simulink model "afe_rst_ctrl"  (R2026b)
settings: Solver=ode23t  StopTime=param.sim.simlength  FixedStep=tc  MaxStep=param.glb_time.tc  RelTol=1e-4
values from neighbouring files (symbols this model uses):
  param = add_template_extras(param, options)    [init_model.m]
undefined symbols (not defined in the file or in its folder): magnitude
libraries: fl_lib x181, nesl_utility x97, igbt_simple_2th_lib x6, afe_uvw_ctrl x5, discrete_time_low_pass_filter x2, threephase_inductor_lib x1, dclink_for_two_levels x1, three_phase_pwm_modulator x1, three_phase_inverter_ideal_switch_based_model x1, three_phase_inverter_mosfet_based_with_thermal_model x1, ee_lib x1, three_phase_voltage_with_frt_emulator_mfcn x1
(part 2 of 6)

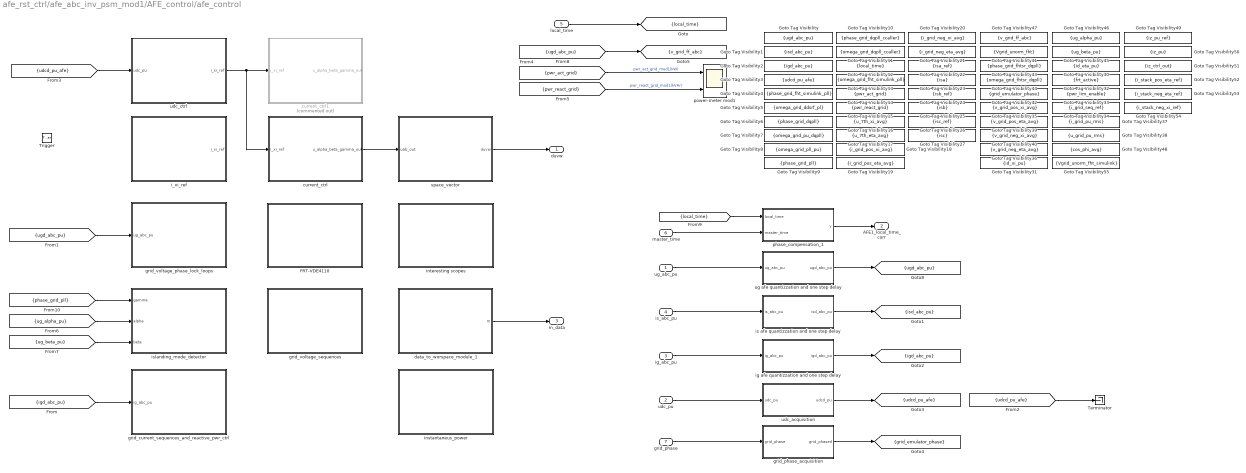
== system afe_rst_ctrl/afe_abc_inv_psm_mod1/AFE_control/afe_control ==
  ug_abc_pu : Inport
  udc_pu : Inport  Port=2
  ig_abc_pu : Inport  Port=3
  is_abc_pu : Inport  Port=4
  local_time : Inport  Port=5
  master_time : Inport  Port=6
  grid_phase : Inport  Port=7
  Trigger : TriggerPort  VariantControl=(inherit)  PortDimensions=1
  FRT-VDE4110 : Subsystem
  Goto Tag Visibility : GotoTagVisibility  GotoTag=ugd_abc_pu
  Goto Tag Visibility1 : GotoTagVisibility  GotoTag=isd_abc_pu
  Goto Tag Visibility10 : GotoTagVisibility  GotoTag=phase_grid_dqpll_ccaller
  Goto Tag Visibility11 : GotoTagVisibility  GotoTag=omega_grid_dqpll_ccaller
  Goto Tag Visibility12 : GotoTagVisibility  GotoTag=local_time
  Goto Tag Visibility13 : GotoTagVisibility  GotoTag=omega_grid_fht_simulink_pll
  Goto Tag Visibility14 : GotoTagVisibility  GotoTag=pwr_act_grid
  Goto Tag Visibility15 : GotoTagVisibility  GotoTag=pwr_react_grid
  Goto Tag Visibility16 : GotoTagVisibility  GotoTag=u_7th_xi_avg
  Goto Tag Visibility17 : GotoTagVisibility  GotoTag=u_7th_eta_avg
  Goto Tag Visibility18 : GotoTagVisibility  GotoTag=i_grid_pos_xi_avg
  Goto Tag Visibility19 : GotoTagVisibility  GotoTag=i_grid_pos_eta_avg
  Goto Tag Visibility2 : GotoTagVisibility  GotoTag=igd_abc_pu
  Goto Tag Visibility20 : GotoTagVisibility  GotoTag=i_grid_neg_xi_avg
  Goto Tag Visibility21 : GotoTagVisibility  GotoTag=i_grid_neg_eta_avg
  Goto Tag Visibility22 : GotoTagVisibility  GotoTag=isa_ref
  Goto Tag Visibility23 : GotoTagVisibility  GotoTag=isa
  Goto Tag Visibility24 : GotoTagVisibility  GotoTag=isb_ref
  Goto Tag Visibility25 : GotoTagVisibility  GotoTag=isb
  Goto Tag Visibility26 : GotoTagVisibility  GotoTag=isc_ref
  Goto Tag Visibility27 : GotoTagVisibility  GotoTag=isc
  Goto Tag Visibility3 : GotoTagVisibility  GotoTag=udcd_pu_afe
  Goto Tag Visibility30 : GotoTagVisibility  GotoTag=id_eta_pu
  Goto Tag Visibility31 : GotoTagVisibility  GotoTag=id_xi_pu
  Goto Tag Visibility32 : GotoTagVisibility  GotoTag=frt_active
  Goto Tag Visibility33 : GotoTagVisibility  GotoTag=pwr_lim_enable
  Goto Tag Visibility34 : GotoTagVisibility  GotoTag=i_grid_seq_ref
  Goto Tag Visibility35 : GotoTagVisibility  GotoTag=v_grid_pos_xi_avg
  Goto Tag Visibility36 : GotoTagVisibility  GotoTag=v_grid_neg_eta_avg
  Goto Tag Visibility37 : GotoTagVisibility  GotoTag=i_grid_pu_rms
  Goto Tag Visibility38 : GotoTagVisibility  GotoTag=u_grid_pu_rms
  Goto Tag Visibility39 : GotoTagVisibility  GotoTag=v_grid_pos_eta_avg
  Goto Tag Visibility4 : GotoTagVisibility  GotoTag=phase_grid_fht_simulink_pll
  Goto Tag Visibility40 : GotoTagVisibility  GotoTag=v_grid_neg_xi_avg
  Goto Tag Visibility41 : GotoTagVisibility  GotoTag=Vgrid_unorm_fht
  Goto Tag Visibility42 : GotoTagVisibility  GotoTag=grid_emulator_phase
  Goto Tag Visibility43 : GotoTagVisibility  GotoTag=phase_grid_fhtsr_dqpll
  Goto Tag Visibility44 : GotoTagVisibility  GotoTag=omega_grid_fhtsr_dqpll
  Goto Tag Visibility45 : GotoTagVisibility  GotoTag=ug_beta_pu
  Goto Tag Visibility46 : GotoTagVisibility  GotoTag=ug_alpha_pu
  Goto Tag Visibility47 : GotoTagVisibility  GotoTag=v_grid_ff_abc
  Goto Tag Visibility48 : GotoTagVisibility  GotoTag=cos_phi_avg
  Goto Tag Visibility49 : GotoTagVisibility  GotoTag=iz_pu_ref
  Goto Tag Visibility5 : GotoTagVisibility  GotoTag=omega_grid_ddsrf_pl
  Goto Tag Visibility50 : GotoTagVisibility  GotoTag=iz_pu
  Goto Tag Visibility51 : GotoTagVisibility  GotoTag=iz_ctrl_out
  Goto Tag Visibility52 : GotoTagVisibility  GotoTag=i_stack_pos_eta_ref
  Goto Tag Visibility53 : GotoTagVisibility  GotoTag=i_stack_neg_eta_ref
  Goto Tag Visibility54 : GotoTagVisibility  GotoTag=i_stack_neg_xi_ref
  Goto Tag Visibility55 : GotoTagVisibility  GotoTag=Vgrid_unorm_fht_simulink
  Goto Tag Visibility6 : GotoTagVisibility  GotoTag=phase_grid_dqpll
  Goto Tag Visibility7 : GotoTagVisibility  GotoTag=omega_grid_pu_dqpll
  Goto Tag Visibility8 : GotoTagVisibility  GotoTag=omega_grid_pll_pu
  Goto Tag Visibility9 : GotoTagVisibility  GotoTag=phase_grid_pll
  Terminator : Terminator
  current_ctrl : Subsystem
  current_ctrl1 : Subsystem  Commented=on
  data_to_worspace_module_1 : Subsystem
  grid_current_sequences_and_reactive_pwr_ctrl : Subsystem
  grid_phase_acquisition : Subsystem
  grid_voltage_phase_lock_loops : Subsystem
  grid_voltage_sequences : Subsystem
  i_xi_ref : Subsystem
  ig afe quantizzation and one step delay : Subsystem
  instantaneus_power : Subsystem
  interesting scopes : Subsystem
  is afe quantizzation and one step delay : Subsystem
  islanding_mode_detector : Subsystem
  phase_compensation_1 : Subsystem
  power-meter mod1 : Scope  NumInputPorts=2
      settings: ActiveDisplayYMinimum=-67.030069207436668  ActiveDisplayYMaximum=116.57466656594397  DataLoggingVariableName=ScopeData9
  space_vector : Subsystem
  udc_acquisition : Subsystem
  udc_ctrl : Subsystem
  ug afe quantizzation and one step delay : Subsystem
  duvw : Outport
  AFE1_local_time_corr : Outport  Port=2
  m_data : Outport  Port=3
  tag scope: grid_emulator_phase=scoped, igd_abc_pu=scoped, isd_abc_pu=scoped, local_time=scoped, udcd_pu_afe=scoped, ugd_abc_pu=scoped, v_grid_ff_abc=scoped
  wires:
  ug_abc_pu/1 -> ug afe quantizzation and one step delay/1(ug_abc_pu)
  space_vector/1(duvw) -> duvw/1
  is_abc_pu/1 -> is afe quantizzation and one step delay/1(is_abc_pu)
  ig_abc_pu/1 -> ig afe quantizzation and one step delay/1(ig_abc_pu)
  [ugd_abc_pu] -> grid_voltage_phase_lock_loops/1(ug_abc_pu)
  [igd_abc_pu] -> grid_current_sequences_and_reactive_pwr_ctrl/1(ig_abc_pu)
  [udcd_pu_afe] -> udc_ctrl/1(udc_pu)
  udc_pu/1 -> udc_acquisition/1(udc_pu)
  udc_acquisition/1(udcd_pu) -> [udcd_pu_afe]
  [pwr_react_grid] -> power-meter mod1/2  "pwr_react_grid_mod1(kVAr)"
  [pwr_act_grid] -> power-meter mod1/1  "pwr_act_grid_mod1(kW)"
  [phase_grid_pll] -> islanding_mode_detector/1(gamma)
  [ug_alpha_pu] -> islanding_mode_detector/2(alpha)
  ug afe quantizzation and one step delay/1(ugd_abc_pu) -> [ugd_abc_pu]
  is afe quantizzation and one step delay/1(isd_abc_pu) -> [isd_abc_pu]
  ig afe quantizzation and one step delay/1(igd_abc_pu) -> [igd_abc_pu]
  [ug_beta_pu] -> islanding_mode_detector/3(beta)
  local_time/1 -> [local_time]
  master_time/1 -> phase_compensation_1/2(master_time)
  phase_compensation_1/1(y) -> AFE1_local_time_corr/1
  [local_time] -> phase_compensation_1/1(local_time)
  grid_phase/1 -> grid_phase_acquisition/1(grid_phase)
  grid_phase_acquisition/1(grid_phased) -> [grid_emulator_phase]
  [ugd_abc_pu] -> [v_grid_ff_abc]
  data_to_worspace_module_1/1(m) -> m_data/1
  [udcd_pu_afe] -> Terminator/1
  udc_ctrl/1(i_xi_ref) -> current_ctrl/1(i_xi_ref), current_ctrl1/1(i_xi_ref)
  current_ctrl/1(u_alpha_beta_gamma_out) -> space_vector/1(uab_out)

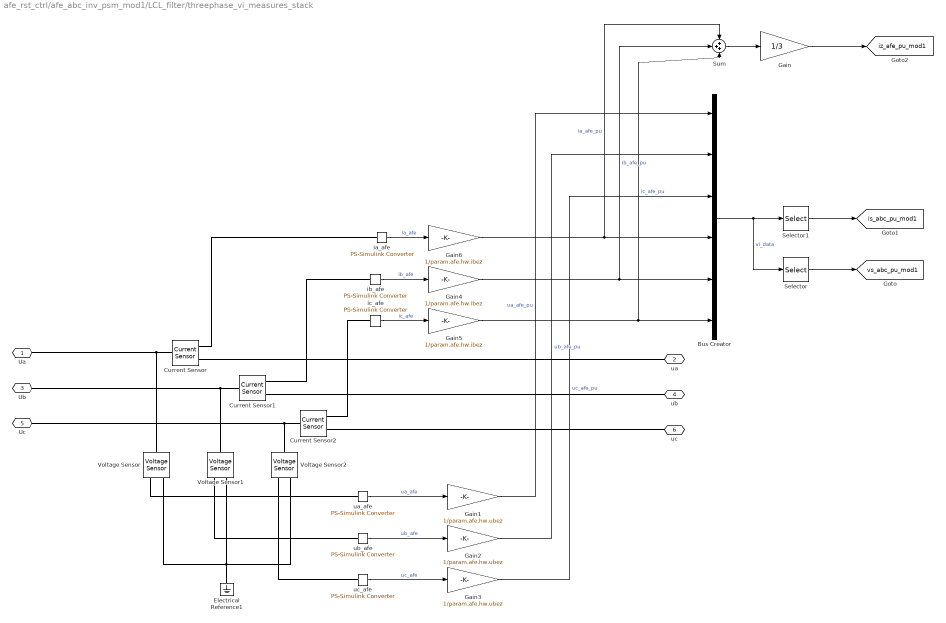
== system afe_rst_ctrl/afe_abc_inv_psm_mod1/LCL_filter/threephase_vi_measures_stack ==
  Bus Creator : BusCreator  Inputs=6
  Current Sensor : fl_lib/Electrical/Electrical Sensors/Current Sensor
  Current Sensor1 : fl_lib/Electrical/Electrical Sensors/Current Sensor
  Current Sensor2 : fl_lib/Electrical/Electrical Sensors/Current Sensor
  Electrical Reference1 : fl_lib/Electrical/Electrical Elements/Electrical Reference
  Gain : Gain  Gain=1/3
  Gain1 : Gain  Gain=1/param.afe.hw.ubez
  Gain2 : Gain  Gain=1/param.afe.hw.ubez
  Gain3 : Gain  Gain=1/param.afe.hw.ubez
  Gain4 : Gain  Gain=1/param.afe.hw.ibez
  Gain5 : Gain  Gain=1/param.afe.hw.ibez
  Gain6 : Gain  Gain=1/param.afe.hw.ibez
  Selector : Selector  InputPortWidth=6  IndexOptions=Index vector (dialog)  Indices=[1 2 3]  OutputSizes=1  RuntimeRangeChecks=off
  Selector1 : Selector  InputPortWidth=6  IndexOptions=Index vector (dialog)  Indices=[4 5 6]  OutputSizes=1  RuntimeRangeChecks=off
  Sum : Sum  Inputs=+++
  Voltage Sensor : fl_lib/Electrical/Electrical Sensors/Voltage Sensor
  Voltage Sensor1 : fl_lib/Electrical/Electrical Sensors/Voltage Sensor
  Voltage Sensor2 : fl_lib/Electrical/Electrical Sensors/Voltage Sensor
  ia_afe : nesl_utility/PS-Simulink Converter  PhysicalDomain=network_engine_domain  SubClassName=ps_output  LeftPortType=input  RightPortType=output  PseudoPeriodic=off  Frequencies=[]  VectorFormat=1-D array  Unit=A  AffineConversion=off
  ib_afe : nesl_utility/PS-Simulink Converter  PhysicalDomain=network_engine_domain  SubClassName=ps_output  LeftPortType=input  RightPortType=output  PseudoPeriodic=off  Frequencies=[]  VectorFormat=1-D array  Unit=A  AffineConversion=off
  ic_afe : nesl_utility/PS-Simulink Converter  PhysicalDomain=network_engine_domain  SubClassName=ps_output  LeftPortType=input  RightPortType=output  PseudoPeriodic=off  Frequencies=[]  VectorFormat=1-D array  Unit=A  AffineConversion=off
  ua_afe : nesl_utility/PS-Simulink Converter  PhysicalDomain=network_engine_domain  SubClassName=ps_output  LeftPortType=input  RightPortType=output  PseudoPeriodic=off  Frequencies=[]  VectorFormat=1-D array  Unit=V  AffineConversion=off
  ub_afe : nesl_utility/PS-Simulink Converter  PhysicalDomain=network_engine_domain  SubClassName=ps_output  LeftPortType=input  RightPortType=output  PseudoPeriodic=off  Frequencies=[]  VectorFormat=1-D array  Unit=V  AffineConversion=off
  uc_afe : nesl_utility/PS-Simulink Converter  PhysicalDomain=network_engine_domain  SubClassName=ps_output  LeftPortType=input  RightPortType=output  PseudoPeriodic=off  Frequencies=[]  VectorFormat=1-D array  Unit=V  AffineConversion=off
  Ua : PMIOPort  Side=Left
  ua : PMIOPort  Port=2  Side=Right
  Ub : PMIOPort  Port=3  Side=Left
  ub : PMIOPort  Port=4  Side=Right
  Uc : PMIOPort  Port=5  Side=Left
  uc : PMIOPort  Port=6  Side=Right
  tag scope: is_abc_pu_mod1=global, iz_afe_pu_mod1=global, vs_abc_pu_mod1=global
  wires:
  Bus Creator/1 -> Selector/1, Selector1/1  "vi_data"
  Selector/1 -> [vs_abc_pu_mod1]
  ib_afe/1 -> Gain4/1  "ib_afe"
  ia_afe/1 -> Gain6/1  "ia_afe"
  ic_afe/1 -> Gain5/1  "ic_afe"
  ua_afe/1 -> Gain1/1  "ua_afe"
  ub_afe/1 -> Gain2/1  "ub_afe"
  uc_afe/1 -> Gain3/1  "uc_afe"
  Selector1/1 -> [is_abc_pu_mod1]
  Sum/1 -> Gain/1
  Gain/1 -> [iz_afe_pu_mod1]
  Gain1/1 -> Bus Creator/1  "ua_afe_pu"
  Gain2/1 -> Bus Creator/2  "ub_afe_pu"
  Gain3/1 -> Bus Creator/3  "uc_afe_pu"
  Gain6/1 -> Sum/1, Bus Creator/4  "ia_afe_pu"
  Gain4/1 -> Sum/2, Bus Creator/5  "ib_afe_pu"
  Gain5/1 -> Bus Creator/6, Sum/3  "ic_afe_pu"
  connections:
  Current Sensor1/LConn1 -- Ub/RConn1 -- Voltage Sensor1/LConn1
  Electrical Reference1/LConn1 -- Voltage Sensor/RConn2 -- Voltage Sensor2/RConn2 -- Voltage Sensor1/RConn2
  Voltage Sensor/RConn1 -- ua_afe/LConn1
  Current Sensor/RConn2 -- ua/RConn1
  Voltage Sensor1/RConn1 -- ub_afe/LConn1
  Voltage Sensor2/LConn1 -- Uc/RConn1 -- Current Sensor2/LConn1
  Current Sensor/LConn1 -- Ua/RConn1 -- Voltage Sensor/LConn1
  Current Sensor1/RConn2 -- ub/RConn1
  Voltage Sensor2/RConn1 -- uc_afe/LConn1
  ib_afe/LConn1 -- Current Sensor1/RConn1
  ia_afe/LConn1 -- Current Sensor/RConn1
  ic_afe/LConn1 -- Current Sensor2/RConn1
  Current Sensor2/RConn2 -- uc/RConn1

== system afe_rst_ctrl/afe_abc_inv_psm_mod1/LCL_filter/threephase_vi_measures_stack1 ==
  Bus Creator : BusCreator  Inputs=6
  Current Sensor : fl_lib/Electrical/Electrical Sensors/Current Sensor
  Current Sensor1 : fl_lib/Electrical/Electrical Sensors/Current Sensor
  Current Sensor2 : fl_lib/Electrical/Electrical Sensors/Current Sensor
  Electrical Reference1 : fl_lib/Electrical/Electrical Elements/Electrical Reference
  Gain1 : Gain  Gain=1/param.afe.hw.ubez
  Gain2 : Gain  Gain=1/param.afe.hw.ubez
  Gain3 : Gain  Gain=1/param.afe.hw.ubez
  Gain4 : Gain  Gain=1/param.afe.hw.ibez
  Gain5 : Gain  Gain=1/param.afe.hw.ibez
  Gain6 : Gain  Gain=1/param.afe.hw.ibez
  Selector : Selector  InputPortWidth=6  IndexOptions=Index vector (dialog)  Indices=[1 2 3]  OutputSizes=1  RuntimeRangeChecks=off
  Selector1 : Selector  InputPortWidth=6  IndexOptions=Index vector (dialog)  Indices=[4 5 6]  OutputSizes=1  RuntimeRangeChecks=off
  Voltage Sensor : fl_lib/Electrical/Electrical Sensors/Voltage Sensor
  Voltage Sensor1 : fl_lib/Electrical/Electrical Sensors/Voltage Sensor
  Voltage Sensor2 : fl_lib/Electrical/Electrical Sensors/Voltage Sensor
  ia_grid : nesl_utility/PS-Simulink Converter  PhysicalDomain=network_engine_domain  SubClassName=ps_output  LeftPortType=input  RightPortType=output  PseudoPeriodic=off  Frequencies=[]  VectorFormat=1-D array  Unit=A  AffineConversion=off
  ib_grid : nesl_utility/PS-Simulink Converter  PhysicalDomain=network_engine_domain  SubClassName=ps_output  LeftPortType=input  RightPortType=output  PseudoPeriodic=off  Frequencies=[]  VectorFormat=1-D array  Unit=A  AffineConversion=off
  ic_grid : nesl_utility/PS-Simulink Converter  PhysicalDomain=network_engine_domain  SubClassName=ps_output  LeftPortType=input  RightPortType=output  PseudoPeriodic=off  Frequencies=[]  VectorFormat=1-D array  Unit=A  AffineConversion=off
  ua_grid : nesl_utility/PS-Simulink Converter  PhysicalDomain=network_engine_domain  SubClassName=ps_output  LeftPortType=input  RightPortType=output  PseudoPeriodic=off  Frequencies=[]  VectorFormat=1-D array  Unit=V  AffineConversion=off
  ub_grid : nesl_utility/PS-Simulink Converter  PhysicalDomain=network_engine_domain  SubClassName=ps_output  LeftPortType=input  RightPortType=output  PseudoPeriodic=off  Frequencies=[]  VectorFormat=1-D array  Unit=V  AffineConversion=off
  uc_grid : nesl_utility/PS-Simulink Converter  PhysicalDomain=network_engine_domain  SubClassName=ps_output  LeftPortType=input  RightPortType=output  PseudoPeriodic=off  Frequencies=[]  VectorFormat=1-D array  Unit=V  AffineConversion=off
  Ua : PMIOPort  Side=Left
  ua : PMIOPort  Port=2  Side=Right
  Ub : PMIOPort  Port=3  Side=Left
  ub : PMIOPort  Port=4  Side=Right
  Uc : PMIOPort  Port=5  Side=Left
  uc : PMIOPort  Port=6  Side=Right
  tag scope: ig_abc_pu_mod1=global, ug_abc_pu_mod1=global
  wires:
  Selector1/1 -> [ig_abc_pu_mod1]
  uc_grid/1 -> Gain3/1
  ub_grid/1 -> Gain2/1
  ua_grid/1 -> Gain1/1
  ic_grid/1 -> Gain5/1
  ia_grid/1 -> Gain6/1
  ib_grid/1 -> Gain4/1
  Selector/1 -> [ug_abc_pu_mod1]
  Bus Creator/1 -> Selector1/1, Selector/1  "vi_data"
  Gain1/1 -> Bus Creator/1  "ua_grid_pu"
  Gain2/1 -> Bus Creator/2  "ub_grid_pu"
  Gain3/1 -> Bus Creator/3  "uc_grid_pu"
  Gain6/1 -> Bus Creator/4  "ia_grid_pu"
  Gain4/1 -> Bus Creator/5  "ib_grid_pu"
  Gain5/1 -> Bus Creator/6  "ic_grid_pu"
  connections:
  Current Sensor2/RConn2 -- uc/RConn1
  ic_grid/LConn1 -- Current Sensor2/RConn1
  ia_grid/LConn1 -- Current Sensor/RConn1
  ib_grid/LConn1 -- Current Sensor1/RConn1
  Voltage Sensor2/RConn1 -- uc_grid/LConn1
  Current Sensor1/RConn2 -- ub/RConn1
  Voltage Sensor/LConn1 -- Current Sensor/LConn1 -- Ua/RConn1
  Current Sensor2/LConn1 -- Voltage Sensor2/LConn1 -- Uc/RConn1
  Voltage Sensor1/RConn1 -- ub_grid/LConn1
  Current Sensor/RConn2 -- ua/RConn1
  Voltage Sensor/RConn1 -- ua_grid/LConn1
  Voltage Sensor1/RConn2 -- Voltage Sensor2/RConn2 -- Voltage Sensor/RConn2 -- Electrical Reference1/LConn1
  Voltage Sensor1/LConn1 -- Current Sensor1/LConn1 -- Ub/RConn1

== system afe_rst_ctrl/afe_abc_inv_psm_mod1/afe/sv_pwm ==
  duties_uvw : Inport
  Bus Selector2 : BusSelector  OutputSignals=du(k),dv(k),dw(k)
  Constant1 : Constant  Value=param.afe.behav.pwm_phase_shift_mod1
  modulator1 : Subsystem
  td2tc_1 : TransferFcn  Denominator=[param.glb_time.tc 1]
  td2tc_2 : TransferFcn  Denominator=[param.glb_time.tc 1]
  td2tc_3 : TransferFcn  Denominator=[param.glb_time.tc 1]
  gate_cmds : Outport
  wires:
  modulator1/1(gate_cmds) -> gate_cmds/1
  Constant1/1 -> modulator1/4(phase)
  Bus Selector2/1 -> td2tc_1/1  "<du(k)>"
  Bus Selector2/2 -> td2tc_2/1  "<dv(k)>"
  Bus Selector2/3 -> td2tc_3/1  "<dw(k)>"
  duties_uvw/1 -> Bus Selector2/1
  td2tc_1/1 -> modulator1/1(u)  "du(t)"
  td2tc_3/1 -> modulator1/3(w)  "dw(t)"
  td2tc_2/1 -> modulator1/2(v)  "dv(t)"

== system afe_rst_ctrl/afe_abc_inv_psm_mod1/afe/three_phase_inverter_ideal_switch_based_model ==
  gate_commands : Inport
  three_phase_inverter_ideal_switch_based_model : three_phase_inverter_ideal_switch_based_model/three phase inverter ideal switch based model  Ron_ideal_switch=param.afe.ideal_switch.Rds_on  Vth=param.afe.ideal_switch.Vth  Vgamma=param.afe.ideal_switch.Vdon_diode  Rdon_diode=param.afe.ideal_switch.Rdon_diode  Csnubber=param.afe.ideal_switch.Csnubber  Rsnubber=param.afe.ideal_switch.Rsnubber
  udc(+) : PMIOPort  Side=Left
  u : PMIOPort  Port=2  Side=Right
  v : PMIOPort  Port=3  Side=Right
  udc(-) : PMIOPort  Port=4  Side=Left
  w : PMIOPort  Port=5  Side=Right
  wires:
  gate_commands/1 -> three_phase_inverter_ideal_switch_based_model/1
  connections:
  three_phase_inverter_ideal_switch_based_model/LConn1 -- udc(+)/RConn1
  three_phase_inverter_ideal_switch_based_model/RConn3 -- w/RConn1
  three_phase_inverter_ideal_switch_based_model/RConn2 -- v/RConn1
  three_phase_inverter_ideal_switch_based_model/LConn2 -- udc(-)/RConn1
  three_phase_inverter_ideal_switch_based_model/RConn1 -- u/RConn1

== system afe_rst_ctrl/afe_abc_inv_psm_mod1/afe/three_phase_inverter_igbt_based_with_thermal_model ==
  gate_commands : Inport
  Bus Selector : BusSelector  OutputSignals=module_1.igbt_ploss_Q2,module_1.igbt_voltage_Q2,module_1.igbt_current_Q2,module_1.igbt_JH_temp_Q2,module_1.igbt_HA_temp_Q2
  Bus Selector1 : BusSelector  OutputSignals=module_1.igbt_ploss_Q1,module_1.igbt_voltage_Q1,module_1.igbt_current_Q1,module_1.igbt_JH_temp_Q1,module_1.igbt_HA_temp_Q1
  Bus Selector2 : BusSelector  OutputSignals=module_2.igbt_ploss_Q3,module_2.igbt_voltage_Q3,module_2.igbt_current_Q3,module_2.igbt_JH_temp_Q3,module_2.igbt_HA_temp_Q3
  Bus Selector3 : BusSelector  OutputSignals=module_1.diode_ploss_Q1,module_1.diode_JH_temp_Q1,module_1.diode_HA_temp_Q1,module_1.diode_current_Q1
  three_phase_inverter_with_igbt_simple_2th : Subsystem  mask{vce_sat_m=param.afe.igbt.Vce_sat, v_gamma_m=param.afe.igbt.Vdon_diode, Vth_gate_m=param.afe.igbt.Vth, Vth_gate_hyst_m=0.85, Eon_m=param.afe.igbt.Eon*1000, Eoff_m=param.afe.igbt.Eoff*1000, Err_m=param.afe.igbt.Erec*1000, Ic_ref_m=param.afe.igbt.Ion_sw_losses, Vdc_ref_m=param.afe.igbt.Voff_sw_losses, Vblock_Errf_m=50, rce_on_m=param.afe.igbt.Rce_on*1000, rd_on_m=param.afe.igbt.Rdon_diode*1000, Gce_off_m=1e-6, time_constant_edge_m=param.glb_time.tc, time_constant_ploss_m=1e3, Csnubber_m=param.afe.igbt.Csnubber, Rsnubber_m=param.afe.igbt.Rsnubber, rth_switch_JH_m=param.afe.igbt.Rth_switch_JH, rth_switch_HA_m=param.thermal.heatsink.Rth_switch_HA, rth_diode_JH_m=param.afe.igbt.Rth_diode_JH, rth_diode_HA_m=param.thermal.heatsink.Rth_diode_HA, JunctionTermalMass_m=param.afe.igbt.JunctionTermalMass, Tambient_m=param.thermal.Tambient, mass_heatsink_m=param.thermal.heatsink.no_weight, specific_heat_m=param.thermal.heatsink.cp}
      mask prompts: vce_sat_m "Collector-emitter on-stage voltage [V]"; v_gamma_m "Diode forward voltage [V]"; Vth_gate_m "Gate-emitter threshold voltage [V]"; Vth_gate_hyst_m "Half hysteresis band for the switching events [V]"; Eon_m "Turn-on energy at Ic_ref, Vdc_ref [mJ]"; Eoff_m "Turn-off energy at Ic_ref, Vdc_ref [mJ]"; Err_m "Reverse recovery energy at Ic_ref, Vdc_ref [mJ]"; Ic_ref_m "Reference current of the energies [A]"; Vdc_ref_m "Reference voltage of the energies [V]"; Vblock_Errf_m "V block Err"; rce_on_m "IGBT on-state series resistance [mOhm]"; rd_on_m "Diode series resistance [mOhm]"; Gce_off_m "Off-state conductance [1/Ohm]"; time_constant_edge_m "Sample&hold time constant (<< on-time) [us]"; time_constant_ploss_m "Loss averaging time constant (2-5 x Tsw) [us]"; Csnubber_m "Csnubber [F]"; Rsnubber_m "Rsnubber [Ohm]"; rth_switch_JH_m "Thermal impedance Junction-heatsink switch [K/W]"; rth_switch_HA_m "Thermal impedance heatsink-ambient switch[K/W]"; rth_diode_JH_m "Thermal impedance Junction-heatsink diode [K/W]"; rth_diode_HA_m "Thermal impedance heatsink-ambient diode [K/W]"; JunctionTermalMass_m "Junction Thermal Mass [J/K]"; Tambient_m "Ambient temperature [degC]"; mass_heatsink_m "Mass heatsink [kg]"; specific_heat_m "Specific heat capacity of the heatsink [J/K/Kg]"
  udc(+) : PMIOPort  Side=Left
  u : PMIOPort  Port=2  Side=Right
  v : PMIOPort  Port=3  Side=Right
  udc(-) : PMIOPort  Port=4  Side=Left
  w : PMIOPort  Port=5  Side=Right
  tag scope: diode_HA_temp_afeQ1=global, diode_JH_temp_afeQ1=global, diode_current_afeQ1=global, diode_ploss_afeQ1=global, igbt_HA_temp_afeQ1=global, igbt_HA_temp_afeQ2=global, igbt_HA_temp_afeQ3=global, igbt_JH_temp_afeQ1=global, igbt_JH_temp_afeQ2=global, igbt_JH_temp_afeQ3=global, igbt_current_afeQ1=global, igbt_current_afeQ2=global, igbt_current_afeQ3=global, igbt_ploss_afeQ1=global, igbt_ploss_afeQ2=global, igbt_ploss_afeQ3=global, igbt_voltage_afeQ1=global, igbt_voltage_afeQ2=global, igbt_voltage_afeQ3=global
  wires:
  gate_commands/1 -> three_phase_inverter_with_igbt_simple_2th/1(gate_commands)
  Bus Selector3/3 -> [diode_HA_temp_afeQ1]  "<diode_HA_temp_Q1>"
  Bus Selector/1 -> [igbt_ploss_afeQ2]  "<igbt_ploss_Q2>"
  Bus Selector3/2 -> [diode_JH_temp_afeQ1]  "<diode_JH_temp_Q1>"
  Bus Selector1/2 -> [igbt_voltage_afeQ1]  "<igbt_voltage_Q1>"
  Bus Selector/2 -> [igbt_voltage_afeQ2]  "<igbt_voltage_Q2>"
  Bus Selector/5 -> [igbt_HA_temp_afeQ2]  "<igbt_HA_temp_Q2>"
  Bus Selector2/5 -> [igbt_HA_temp_afeQ3]  "<igbt_HA_temp_Q3>"
  Bus Selector2/2 -> [igbt_voltage_afeQ3]  "<igbt_voltage_Q3>"
  Bus Selector/4 -> [igbt_JH_temp_afeQ2]  "<igbt_JH_temp_Q2>"
  Bus Selector1/4 -> [igbt_JH_temp_afeQ1]  "<igbt_JH_temp_Q1>"
  Bus Selector3/1 -> [diode_ploss_afeQ1]  "<diode_ploss_Q1>"
  Bus Selector2/4 -> [igbt_JH_temp_afeQ3]  "<igbt_JH_temp_Q3>"
  Bus Selector2/3 -> [igbt_current_afeQ3]  "<igbt_current_Q3>"
  three_phase_inverter_with_igbt_simple_2th/1(m) -> Bus Selector3/1, Bus Selector2/1, Bus Selector/1, Bus Selector1/1
  Bus Selector1/3 -> [igbt_current_afeQ1]  "<igbt_current_Q1>"
  Bus Selector/3 -> [igbt_current_afeQ2]  "<igbt_current_Q2>"
  Bus Selector1/5 -> [igbt_HA_temp_afeQ1]  "<igbt_HA_temp_Q1>"
  Bus Selector2/1 -> [igbt_ploss_afeQ3]  "<igbt_ploss_Q3>"
  Bus Selector1/1 -> [igbt_ploss_afeQ1]  "<igbt_ploss_Q1>"
  Bus Selector3/4 -> [diode_current_afeQ1]  "<diode_current_Q1>"
  connections:
  u/RConn1 -- three_phase_inverter_with_igbt_simple_2th/RConn1
  v/RConn1 -- three_phase_inverter_with_igbt_simple_2th/RConn2
  udc(-)/RConn1 -- three_phase_inverter_with_igbt_simple_2th/LConn2
  udc(+)/RConn1 -- three_phase_inverter_with_igbt_simple_2th/LConn1
  w/RConn1 -- three_phase_inverter_with_igbt_simple_2th/RConn3

== system afe_rst_ctrl/afe_abc_inv_psm_mod1/afe/three_phase_inverter_mosfet_based_with_thermal_model ==
  gate_commands : Inport
  Bus Selector : BusSelector  OutputSignals=mosfet_ploss_Q2,mosfet_voltage_Q2,mosfet_current_Q2,mosfet_JH_temp_Q2,mosfet_HA_temp_Q2
  Bus Selector1 : BusSelector  OutputSignals=mosfet_ploss_Q1,mosfet_voltage_Q1,mosfet_current_Q1,mosfet_JH_temp_Q1,mosfet_HA_temp_Q1
  Bus Selector2 : BusSelector  OutputSignals=mosfet_ploss_Q3,mosfet_voltage_Q3,mosfet_current_Q3,mosfet_JH_temp_Q3,mosfet_HA_temp_Q3
  three phase inverter mosfet based with thermal model : three_phase_inverter_mosfet_based_with_thermal_model/three phase inverter mosfet based with thermal model  mass_heatsink_m=0.2  specific_heat_m=880  rth_mosfet_HA_m=0.02  rth_mosfet_JH_m=0.075  Rds_on_m=0.00185  Vth_m=7.5  Eon_m=0.077  Eoff_m=0.108  Voff_sw_loss_m=1300  Ion_sw_loss_m=1000  Vdon_diode_m=4  Rdon_diode_m=0.00185  JunctionTermalMass_m=2  Tambient_m=40  DThs_init_m=0
  u : PMIOPort  Side=Right
  udc(+) : PMIOPort  Port=2  Side=Left
  v : PMIOPort  Port=3  Side=Right
  udc(-) : PMIOPort  Port=4  Side=Left
  w : PMIOPort  Port=5  Side=Right
  tag scope: mosfet_HA_temp_afeQ1=global, mosfet_HA_temp_afeQ2=global, mosfet_HA_temp_afeQ3=global, mosfet_JH_temp_afeQ1=global, mosfet_JH_temp_afeQ2=global, mosfet_JH_temp_afeQ3=global, mosfet_current_afeQ1=global, mosfet_current_afeQ2=global, mosfet_current_afeQ3=global, mosfet_ploss_afeQ1=global, mosfet_ploss_afeQ2=global, mosfet_ploss_afeQ3=global, mosfet_voltage_afeQ1=global, mosfet_voltage_afeQ2=global, mosfet_voltage_afeQ3=global
  wires:
  gate_commands/1 -> three phase inverter mosfet based with thermal model/1
  three phase inverter mosfet based with thermal model/1 -> Bus Selector/1, Bus Selector2/1, Bus Selector1/1
  Bus Selector2/1 -> [mosfet_ploss_afeQ3]  "<mosfet_ploss_Q3>"
  Bus Selector2/2 -> [mosfet_voltage_afeQ3]  "<mosfet_voltage_Q3>"
  Bus Selector2/3 -> [mosfet_current_afeQ3]  "<mosfet_current_Q3>"
  Bus Selector2/5 -> [mosfet_HA_temp_afeQ3]  "<mosfet_HA_temp_Q3>"
  Bus Selector2/4 -> [mosfet_JH_temp_afeQ3]  "<mosfet_JH_temp_Q3>"
  Bus Selector/1 -> [mosfet_ploss_afeQ2]  "<mosfet_ploss_Q2>"
  Bus Selector/2 -> [mosfet_voltage_afeQ2]  "<mosfet_voltage_Q2>"
  Bus Selector/3 -> [mosfet_current_afeQ2]  "<mosfet_current_Q2>"
  Bus Selector/4 -> [mosfet_JH_temp_afeQ2]  "<mosfet_JH_temp_Q2>"
  Bus Selector/5 -> [mosfet_HA_temp_afeQ2]  "<mosfet_HA_temp_Q2>"
  Bus Selector1/1 -> [mosfet_ploss_afeQ1]  "<mosfet_ploss_Q1>"
  Bus Selector1/2 -> [mosfet_voltage_afeQ1]  "<mosfet_voltage_Q1>"
  Bus Selector1/3 -> [mosfet_current_afeQ1]  "<mosfet_current_Q1>"
  Bus Selector1/4 -> [mosfet_JH_temp_afeQ1]  "<mosfet_JH_temp_Q1>"
  Bus Selector1/5 -> [mosfet_HA_temp_afeQ1]  "<mosfet_HA_temp_Q1>"
  connections:
  three phase inverter mosfet based with thermal model/RConn3 -- w/RConn1
  three phase inverter mosfet based with thermal model/RConn2 -- v/RConn1
  three phase inverter mosfet based with thermal model/LConn1 -- udc(+)/RConn1
  three phase inverter mosfet based with thermal model/LConn2 -- udc(-)/RConn1
  three phase inverter mosfet based with thermal model/RConn1 -- u/RConn1

== system afe_rst_ctrl/afe_abc_inv_psm_mod1/brake/Rbrake ==
  PS-Simulink Converter2 : nesl_utility/PS-Simulink Converter  PhysicalDomain=network_engine_domain  SubClassName=ps_output  LeftPortType=input  RightPortType=output  PseudoPeriodic=off  Frequencies=[]  VectorFormat=1-D array  Unit=degC  AffineConversion=off
  PS-Simulink Converter3 : nesl_utility/PS-Simulink Converter  PhysicalDomain=network_engine_domain  SubClassName=ps_output  LeftPortType=input  RightPortType=output  PseudoPeriodic=off  Frequencies=[]  VectorFormat=1-D array  Unit=W  AffineConversion=off
  Rbrake_thermal : Scope  NumInputPorts=2
      settings: ActiveDisplayYMinimum=-0.005623823950706707  ActiveDisplayYMaximum=0.05061441555636037  DataLoggingVariableName=ScopeData33
  Resistor1 : ee_lib/Passive/Resistor  R=param.afe.hw.Rbrake Ohm  enable_R_tol=ee.enum.toleranceApplication.none  R_tol=5  tol_distribution=ee.enum.toleranceDistribution.uniform  nSigma=4  enable_operating_limits=ee.enum.enable.no  operating_limit_action=ee.enum.passive.reportOpLim.warn  power_rating=1 W  max_working_voltage=100 V  noise_mode=ee.enum.sources.noise.Disabled  Tdevice=25 degC  sample_time=1e-3 s  repeatability=ee.enum.ic.repeatability.notRepeatable  user_seed=0  auto_seed=3499211588  power_derating_T1=70 degC  power_derating_T2=155 degC  operating_temperature_range_vec=[-50, 150] degC  alpha=3.93e-3 1/K  Tmeas=25 degC  thermal_mass=100 J/K  temperature_specify=off  temperature_priority=High  temperature=298.15 K  temperature_nominal_specify=off  temperature_nominal_value=1  temperature_nominal_unit=K
  Tambient : fl_lib/Thermal/Thermal Sources/Temperature Source  temperature=param.thermal.Tambient degC
  Temperature Sensor1 : fl_lib/Thermal/Thermal Sensors/Temperature Sensor  temperature_measure=foundation.enum.MeasurementReference.difference
  To Workspace1 : ToWorkspace  VariableName=RbrakePowerFlow_mod1_sim  SampleTime=param.glb_time.tc
      settings: MaxDataPoints=param.glb_time.Nc
  To Workspace10 : ToWorkspace  VariableName=RbrakeTemperature_mod1_sim  SampleTime=param.glb_time.tc
      settings: MaxDataPoints=param.glb_time.Nc
  heatsink_C : fl_lib/Thermal/Thermal Elements/Thermal Mass  mass_type=foundation.enum.constant_variable.constant  mass=40 kg  sp_heat=505 J/(K*kg)  mass_min=1e-6 kg  num_ports=foundation.enum.numPorts2.one  m_specify=off  m_priority=High  m=1 kg  m_nominal_specify=off  m_nominal_value=1  m_nominal_unit=kg  T_specify=on  T_priority=High  T=param.thermal.DThs_init+param.thermal.Tambient degC  T_nominal_specify=off  T_nominal_value=1  T_nominal_unit=K  Q_specify=off  Q_priority=High  Q=0 W  Q_nominal_specify=off  Q_nominal_value=1  Q_nominal_unit=W
  power_losses_switch : fl_lib/Thermal/Thermal Sensors/Heat Flow Rate Sensor
  switch_heatsink : fl_lib/Thermal/Thermal Elements/Thermal Resistance  resistance=300/48e3 K/W  T_specify=off  T_priority=High  T=0 deltadegC  T_nominal_specify=off  T_nominal_value=1  T_nominal_unit=K  Q_specify=off  Q_priority=None  Q=0 W  Q_nominal_specify=off  Q_nominal_value=1  Q_nominal_unit=W
  A : PMIOPort  Side=Left
  B : PMIOPort  Port=2  Side=Right
  wires:
  PS-Simulink Converter2/1 -> To Workspace10/1, Rbrake_thermal/1  "RbrakeTemperature"
  PS-Simulink Converter3/1 -> To Workspace1/1, Rbrake_thermal/2  "RbrakePowerFlow"
  connections:
  Resistor1/LConn1 -- A/RConn1
  Resistor1/RConn1 -- B/RConn1
  Tambient/LConn1 -- Temperature Sensor1/RConn1 -- switch_heatsink/RConn1
  Temperature Sensor1/LConn1 -- power_losses_switch/RConn2 -- heatsink_C/LConn1 -- switch_heatsink/LConn1
  Temperature Sensor1/RConn2 -- PS-Simulink Converter2/LConn1
  power_losses_switch/LConn1 -- Resistor1/LConn2
  power_losses_switch/RConn1 -- PS-Simulink Converter3/LConn1

== system afe_rst_ctrl/afe_abc_inv_psm_mod1/brake/switch_1 ==
  Capacitor : fl_lib/Electrical/Electrical Elements/Capacitor  c=param.afe.ideal_switch.Csnubber F  r=param.afe.ideal_switch.Rsnubber Ohm  g=0 1/Ohm  i_specify=off  i_priority=None  i=0 A  i_nominal_specify=off  i_nominal_value=1  i_nominal_unit=A  v_specify=off  v_priority=None  v=0 V  v_nominal_specify=off  v_nominal_value=1  v_nominal_unit=V  vc_specify=off  vc_priority=High  vc=0 V  vc_nominal_specify=off  vc_nominal_value=1  vc_nominal_unit=V
  Diode : fl_lib/Electrical/Electrical Elements/Diode  Vf=param.afe.ideal_switch.Vgamma V  Ron=param.afe.ideal_switch.Rdon_diode Ohm  Goff=1e-8 1/Ohm  i_specify=off  i_priority=None  i=0 A  i_nominal_specify=off  i_nominal_value=1  i_nominal_unit=A  v_specify=off  v_priority=None  v=0 V  v_nominal_specify=off  v_nominal_value=1  v_nominal_unit=V
  C : PMIOPort  Side=Left
  E : PMIOPort  Port=2  Side=Right
  connections:
  Diode/LConn1 -- Capacitor/RConn1 -- E/RConn1
  Diode/RConn1 -- C/RConn1 -- Capacitor/LConn1

== system afe_rst_ctrl/afe_abc_inv_psm_mod1/brake/switch_2 ==
  Capacitor : fl_lib/Electrical/Electrical Elements/Capacitor  c=param.afe.ideal_switch.Csnubber F  r=param.afe.ideal_switch.Rsnubber Ohm  g=0 1/Ohm  i_specify=off  i_priority=None  i=0 A  i_nominal_specify=off  i_nominal_value=1  i_nominal_unit=A  v_specify=off  v_priority=None  v=0 V  v_nominal_specify=off  v_nominal_value=1  v_nominal_unit=V  vc_specify=off  vc_priority=High  vc=0 V  vc_nominal_specify=off  vc_nominal_value=1  vc_nominal_unit=V
  Diode : fl_lib/Electrical/Electrical Elements/Diode  Vf=param.afe.ideal_switch.Vgamma V  Ron=param.afe.ideal_switch.Rdon_diode Ohm  Goff=1e-8 1/Ohm  i_specify=off  i_priority=None  i=0 A  i_nominal_specify=off  i_nominal_value=1  i_nominal_unit=A  v_specify=off  v_priority=None  v=0 V  v_nominal_specify=off  v_nominal_value=1  v_nominal_unit=V
  Switch : fl_lib/Electrical/Electrical Elements/Switch  R_closed=param.afe.ideal_switch.Rds_on Ohm  G_open=1e-8 1/Ohm  Threshold=7.5  i_specify=off  i_priority=None  i=0 A  i_nominal_specify=off  i_nominal_value=1  i_nominal_unit=A  v_specify=off  v_priority=None  v=0 V  v_nominal_specify=off  v_nominal_value=1  v_nominal_unit=V
  G : PMIOPort  Side=Left
  C : PMIOPort  Port=2  Side=Left
  E : PMIOPort  Port=3  Side=Right
  connections:
  Switch/RConn2 -- C/RConn1 -- Capacitor/LConn1 -- Diode/RConn1
  Switch/RConn1 -- G/RConn1
  Switch/LConn1 -- E/RConn1 -- Capacitor/RConn1 -- Diode/LConn1

== system afe_rst_ctrl/grid/grid_emulator/3ph_Dyg_ssc ==
  Electrical Reference1 : fl_lib/Electrical/Electrical Elements/Electrical Reference
  PS Terminator : fl_lib/Physical Signals/Sinks/PS Terminator
  PS Terminator1 : fl_lib/Physical Signals/Sinks/PS Terminator
  PS Terminator2 : fl_lib/Physical Signals/Sinks/PS Terminator
  configurable_trafo : SimscapeComponentBlock  Description=Configurable transformer: one or two three-phase primaries (star or delta), secondary three-phase (star or delta, any clock number) or single-phase (turns distribution ws) on a three-limb core. Component configurable_transformer.configurable_transformer (pwr-control/library, foundation/electrical_machines/+configurable_transformer).  SourceFile=configurable_transformer.configurable_transformer  ComponentPath=configurable_transformer.configurable_transformer  ComponentVariants="[\"configurable_transformer.configurable_transformer\"]"  ComponentVariantNames="[\"configurable_transformer\"]"  ClassName=configurable_transformer  SchemaVersion=1  primaries=configurable_transformer.n_primaries.one  conn1=configurable_transformer.connection.delta  conn2=configurable_transformer.connection.star  clock2=0  secondary=configurable_transformer.secondary_winding.star  clock3=param.grid.emu.trafo.pu.clock3  ws=[1, -1, 0]  Sr=param.grid.emu.trafo.pwr_nom A*V  V1=param.grid.emu.trafo.u1_nom V  V2=400 V  V3=param.grid.emu.trafo.u2_nom V  fr=param.grid.emu.trafo.f_nom Hz  r1=param.grid.emu.trafo.pu.r1  l1=param.grid.emu.trafo.pu.l1  r2=0.005  l2=0.030  r3=param.grid.emu.trafo.pu.r3  l3=param.grid.emu.trafo.pu.l3  lm=param.grid.emu.trafo.pu.lm  lm0=param.grid.emu.trafo.pu.lm0  rfe=param.grid.emu.trafo.pu.rfe  i1a_specify=off  i1a_priority=None  i1a=0 A  i1a_nominal_specify=off  i1a_nominal_value=1  i1a_nominal_unit=A  i1b_specify=off  i1b_priority=None  i1b=0 A  i1b_nominal_specify=off  i1b_nominal_value=1  i1b_nominal_unit=A  i1c_specify=off  i1c_priority=None  i1c=0 A  i1c_nominal_specify=off  i1c_nominal_value=1  i1c_nominal_unit=A  i2a_specify=off  i2a_priority=None  i2a=0 A  i2a_nominal_specify=off  i2a_nominal_value=1  i2a_nominal_unit=A  i2b_specify=off  i2b_priority=None  i2b=0 A  i2b_nominal_specify=off  i2b_nominal_value=1  i2b_nominal_unit=A  i2c_specify=off  i2c_priority=None  i2c=0 A  i2c_nominal_specify=off  i2c_nominal_value=1  i2c_nominal_unit=A  i3a_specify=off  i3a_priority=None  i3a=0 A  i3a_nominal_specify=off  i3a_nominal_value=1  i3a_nominal_unit=A  i3b_specify=off  i3b_priority=None  i3b=0 A  i3b_nominal_specify=off  i3b_nominal_value=1  i3b_nominal_unit=A  i3c_specify=off  i3c_priority=None  i3c=0 A  i3c_nominal_specify=off  i3c_nominal_value=1  i3c_nominal_unit=A  i3_specify=off  i3_priority=None  i3=0 A  i3_nominal_specify=off  i3_nominal_value=1  i3_nominal_unit=A
      settings: CopyFcn=simscape.sscblock.internal.componentBlockCallback(gcbh,'COPY')  PreCopyFcn=simscape.sscblock.internal.componentBlockCallback(gcbh,'PRECOPY')  PreDeleteFcn=simscape.sscblock.internal.componentBlockCallback(gcbh,'PREDELETE')
      mask Type: configurable_trafo
  ua : PMIOPort  Side=Right
  ub : PMIOPort  Port=2  Side=Right
  uc : PMIOPort  Port=3  Side=Right
  Ua : PMIOPort  Port=4  Side=Left
  Ub : PMIOPort  Port=5  Side=Left
  Uc : PMIOPort  Port=6  Side=Left
  connections:
  Uc/RConn1 -- configurable_trafo/LConn3
  configurable_trafo/LConn2 -- Ub/RConn1
  configurable_trafo/RConn1 -- ua/RConn1
  configurable_trafo/LConn1 -- Ua/RConn1
  ub/RConn1 -- configurable_trafo/RConn2
  configurable_trafo/RConn3 -- uc/RConn1
  Electrical Reference1/LConn1 -- configurable_trafo/RConn4
  PS Terminator/LConn1 -- configurable_trafo/RConn5
  PS Terminator1/LConn1 -- configurable_trafo/RConn6
  configurable_trafo/RConn7 -- PS Terminator2/LConn1

== system afe_rst_ctrl/grid/grid_emulator/threephase_vi_measures ==
  Bus Creator : BusCreator  Inputs=6
  Current Sensor : fl_lib/Electrical/Electrical Sensors/Current Sensor
  Current Sensor1 : fl_lib/Electrical/Electrical Sensors/Current Sensor
  Current Sensor2 : fl_lib/Electrical/Electrical Sensors/Current Sensor
  Electrical Reference1 : fl_lib/Electrical/Electrical Elements/Electrical Reference
  Voltage Sensor : fl_lib/Electrical/Electrical Sensors/Voltage Sensor
  Voltage Sensor1 : fl_lib/Electrical/Electrical Sensors/Voltage Sensor
  Voltage Sensor2 : fl_lib/Electrical/Electrical Sensors/Voltage Sensor
  i : Selector  InputPortWidth=6  IndexOptions=Index vector (dialog)  Indices=[4 5 6]  OutputSizes=1  RuntimeRangeChecks=off
  ia_grid : nesl_utility/PS-Simulink Converter  PhysicalDomain=network_engine_domain  SubClassName=ps_output  LeftPortType=input  RightPortType=output  PseudoPeriodic=off  Frequencies=[]  VectorFormat=1-D array  Unit=A  AffineConversion=off
  ib_grid : nesl_utility/PS-Simulink Converter  PhysicalDomain=network_engine_domain  SubClassName=ps_output  LeftPortType=input  RightPortType=output  PseudoPeriodic=off  Frequencies=[]  VectorFormat=1-D array  Unit=A  AffineConversion=off
  ic_grid : nesl_utility/PS-Simulink Converter  PhysicalDomain=network_engine_domain  SubClassName=ps_output  LeftPortType=input  RightPortType=output  PseudoPeriodic=off  Frequencies=[]  VectorFormat=1-D array  Unit=A  AffineConversion=off
  u : Selector  InputPortWidth=6  IndexOptions=Index vector (dialog)  Indices=[1 2 3]  OutputSizes=1  RuntimeRangeChecks=off
  ua_grid : nesl_utility/PS-Simulink Converter  PhysicalDomain=network_engine_domain  SubClassName=ps_output  LeftPortType=input  RightPortType=output  PseudoPeriodic=off  Frequencies=[]  VectorFormat=1-D array  Unit=V  AffineConversion=off
  ub_grid : nesl_utility/PS-Simulink Converter  PhysicalDomain=network_engine_domain  SubClassName=ps_output  LeftPortType=input  RightPortType=output  PseudoPeriodic=off  Frequencies=[]  VectorFormat=1-D array  Unit=V  AffineConversion=off
  uc_grid : nesl_utility/PS-Simulink Converter  PhysicalDomain=network_engine_domain  SubClassName=ps_output  LeftPortType=input  RightPortType=output  PseudoPeriodic=off  Frequencies=[]  VectorFormat=1-D array  Unit=V  AffineConversion=off
  Ua : PMIOPort  Side=Left
  ua : PMIOPort  Port=2  Side=Right
  Ub : PMIOPort  Port=3  Side=Left
  ub : PMIOPort  Port=4  Side=Right
  Uc : PMIOPort  Port=5  Side=Left
  uc : PMIOPort  Port=6  Side=Right
  tag scope: i_abc_line=global, u_abc_line=global
  wires:
  Bus Creator/1 -> i/1, u/1  "vi_data"
  ib_grid/1 -> Bus Creator/5  "ib"
  ia_grid/1 -> Bus Creator/4  "ia"
  ic_grid/1 -> Bus Creator/6  "ic"
  ua_grid/1 -> Bus Creator/1  "ua"
  ub_grid/1 -> Bus Creator/2  "ub"
  uc_grid/1 -> Bus Creator/3  "uc"
  i/1 -> [i_abc_line]
  u/1 -> [u_abc_line]
  connections:
  Current Sensor1/LConn1 -- Ub/RConn1 -- Voltage Sensor1/LConn1
  Electrical Reference1/LConn1 -- Voltage Sensor/RConn2 -- Voltage Sensor2/RConn2 -- Voltage Sensor1/RConn2
  Voltage Sensor/RConn1 -- ua_grid/LConn1
  Current Sensor/RConn2 -- ua/RConn1
  Voltage Sensor1/RConn1 -- ub_grid/LConn1
  Voltage Sensor2/LConn1 -- Current Sensor2/LConn1 -- Uc/RConn1
  Current Sensor/LConn1 -- Ua/RConn1 -- Voltage Sensor/LConn1
  Current Sensor1/RConn2 -- ub/RConn1
  Voltage Sensor2/RConn1 -- uc_grid/LConn1
  ib_grid/LConn1 -- Current Sensor1/RConn1
  ia_grid/LConn1 -- Current Sensor/RConn1
  ic_grid/LConn1 -- Current Sensor2/RConn1
  Current Sensor2/RConn2 -- uc/RConn1

== system afe_rst_ctrl/afe_abc_inv_psm_mod1/AFE_control/afe_control/FRT-VDE4110 ==
  Constant4 : Constant  Value=0
  Mux : Mux
  Mux1 : Mux  Inputs=2
  enable : Step  Time=param.frt.data.settle_time  FinalValue=param.frt.data.enable_frt_1 + param.frt.data.enable_frt_2
  frt_detection_output : Scope  NumInputPorts=3
      settings: ActiveDisplayYMinimum=-0.12499999999999997  ActiveDisplayYMaximum=1.125
  frt_vde4110 : afe_uvw_ctrl/frt_vde4110  p=param.afe.uvw
  positive_reactive_current_reference : Subsystem
  reset : Step  Time=0.025  InitialValue=1  FinalValue=0
  tag scope: frt_active=scoped, i_grid_seq_ref=scoped, pwr_lim_enable=scoped
  wires:
  frt_vde4110/2 -> [frt_active], frt_detection_output/2  "frt_active"
  frt_vde4110/3 -> [pwr_lim_enable], frt_detection_output/3  "pwr_lim_enable"
  frt_vde4110/4 -> frt_detection_output/1  "frt_state"
  reset/1 -> frt_vde4110/4  "reset"
  enable/1 -> frt_vde4110/3  "enable"
  [v_grid_neg_eta_avg] -> Mux/4
  [v_grid_neg_xi_avg] -> Mux/3
  [v_grid_pos_eta_avg] -> Mux/2
  [v_grid_pos_xi_avg] -> Mux/1
  Mux/1 -> frt_vde4110/1
  positive_reactive_current_reference/1(i_react_pos_ref) -> [i_react_pos_ref]
  Constant4/1 -> [i_react_neg_ref]
  frt_vde4110/1 -> [i_grid_seq_ref]
  [i_react_neg_ref] -> Mux1/2
  [i_react_pos_ref] -> Mux1/1
  Mux1/1 -> frt_vde4110/2

== system afe_rst_ctrl/afe_abc_inv_psm_mod1/AFE_control/afe_control/current_ctrl ==
  i_xi_ref : Inport
  Mux : Mux  Inputs=3
  current_ctrl_uvw : afe_uvw_ctrl/current_ctrl_uvw  p=param.afe.uvw
  isa_ref/isa : Scope  NumInputPorts=2
      settings: ActiveDisplayYMinimum=-3.5647345146351177  ActiveDisplayYMaximum=2.2290599372806974
  u_alpha_beta_gamma_out : Outport
  wires:
  i_xi_ref/1 -> current_ctrl_uvw/1  "is_pos_xi_ref"
  [i_stack_neg_xi_ref] -> Mux/2  "is_neg_xi_ref"
  [i_stack_pos_eta_ref] -> Mux/1  "is_pos_eta_ref"
  [i_stack_neg_eta_ref] -> Mux/3  "is_neg_eta_ref"
  [phase_grid_pll] -> current_ctrl_uvw/4
  [isd_abc_pu] -> current_ctrl_uvw/3
  current_ctrl_uvw/1 -> u_alpha_beta_gamma_out/1
  current_ctrl_uvw/2 -> isa_ref/isa/1
  current_ctrl_uvw/3 -> isa_ref/isa/2
  Mux/1 -> current_ctrl_uvw/2

== system afe_rst_ctrl/afe_abc_inv_psm_mod1/AFE_control/afe_control/current_ctrl1 ==
  i_xi_ref : Inport
  Demux : Demux  Outputs=3
  current_transformation : Subsystem
  inner_current_ctrl : Subsystem
  xieta2abc_ref : Subsystem
  u_alpha_beta_gamma_out : Outport
  wires:
  Demux/1 -> current_transformation/1(is_a_pu)  "is_a"
  Demux/2 -> current_transformation/2(is_b_pu)  "is_b"
  Demux/3 -> current_transformation/3(is_c_pu)  "is_c"
  [isd_abc_pu] -> Demux/1
  [phase_grid_pll] -> xieta2abc_ref/5(phase)
  xieta2abc_ref/1(i_abc_ref) -> inner_current_ctrl/1(In1)
  [isd_abc_pu] -> inner_current_ctrl/2(is_abc)
  inner_current_ctrl/1(uabg) -> u_alpha_beta_gamma_out/1
  i_xi_ref/1 -> xieta2abc_ref/1(pos_xi_ref)  "i_xi_ref"
  [i_stack_neg_eta_ref] -> xieta2abc_ref/4(neg_eta)
  [i_stack_neg_xi_ref] -> xieta2abc_ref/3(neg_xi)
  [i_stack_pos_eta_ref] -> xieta2abc_ref/2(pos_eta)

== system afe_rst_ctrl/afe_abc_inv_psm_mod1/AFE_control/afe_control/data_to_worspace_module_1 ==
  Bus Creator : BusCreator  Inputs=5
  dq_pll : Subsystem
  inner_current_tracking : Subsystem
  pwr_meter : Subsystem
  sequences_data : Subsystem
  m : Outport
  wires:
  Bus Creator/1 -> m/1
  sequences_data/1(m_seq) -> Bus Creator/1  "sequences_data"
  pwr_meter/1(m_pwr_meter) -> Bus Creator/2  "pwr_meter"
  inner_current_tracking/1(m_inner_current_tracking) -> Bus Creator/3  "m_inner_current_tracking"
  [local_time] -> Bus Creator/5  "local_time"
  dq_pll/1(dqPLLs) -> Bus Creator/4  "dq_pll"

== system afe_rst_ctrl/afe_abc_inv_psm_mod1/AFE_control/afe_control/grid_current_sequences_and_reactive_pwr_ctrl ==
  ig_abc_pu : Inport
  Abs : Abs  SaturateOnIntegerOverflow=off
  Demux : Demux  Outputs=3
  Demux1 : Demux
  Saturation : Saturate  UpperLimit=2  LowerLimit=0.1
  Terminator : Terminator
  grid_current_sequences_q_ctrl : afe_uvw_ctrl/grid_current_sequences_q_ctrl  p=param.afe.uvw
  tag scope: i_grid_neg_eta_avg=scoped, i_grid_neg_xi_avg=scoped, i_grid_pos_eta_avg=scoped, i_grid_pos_xi_avg=scoped, i_stack_neg_eta_ref=scoped, i_stack_neg_xi_ref=scoped, i_stack_pos_eta_ref=scoped
  wires:
  [phase_grid_pll] -> grid_current_sequences_q_ctrl/2
  ig_abc_pu/1 -> grid_current_sequences_q_ctrl/1
  grid_current_sequences_q_ctrl/1 -> Demux/1
  Demux/1 -> [i_stack_pos_eta_ref]
  grid_current_sequences_q_ctrl/2 -> Demux1/1
  Demux1/1 -> [i_grid_pos_xi_avg]
  Demux1/2 -> [i_grid_pos_eta_avg]
  Demux1/3 -> [i_grid_neg_xi_avg]
  Demux1/4 -> [i_grid_neg_eta_avg]
  grid_current_sequences_q_ctrl/3 -> Terminator/1
  [i_grid_seq_ref] -> grid_current_sequences_q_ctrl/4
  Saturation/1 -> grid_current_sequences_q_ctrl/3
  [omega_grid_pll_pu] -> Abs/1
  Abs/1 -> Saturation/1
  Demux/2 -> [i_stack_neg_xi_ref]
  Demux/3 -> [i_stack_neg_eta_ref]

== system afe_rst_ctrl/afe_abc_inv_psm_mod1/AFE_control/afe_control/grid_phase_acquisition ==
  grid_phase : Inport
  Quantizer : Quantizer  QuantizationInterval=param.meas.adc_quantization
  Unit Delay : UnitDelay  SampleTime=-1
  Zero-Order Hold : ZeroOrderHold  SampleTime=-1
  grid_phased : Outport
  wires:
  Zero-Order Hold/1 -> Quantizer/1
  Unit Delay/1 -> grid_phased/1
  grid_phase/1 -> Zero-Order Hold/1
  Quantizer/1 -> Unit Delay/1

== system afe_rst_ctrl/afe_abc_inv_psm_mod1/AFE_control/afe_control/grid_voltage_phase_lock_loops ==
  ug_abc_pu : Inport
  Bus Creator2 : BusCreator  Inputs=2
  FHT-PLL performance : Scope  NumInputPorts=2
      settings: ActiveDisplayYMinimum=-1.32501220703125  ActiveDisplayYMaximum=1.30987548828125  DataLoggingVariableName=ScopeData8
  FHT-PLL_simulink : Subsystem
  tag scope: omega_grid_pll_pu=scoped, phase_grid_pll=scoped
  wires:
  FHT-PLL_simulink/1(gamma_grid_fht_pll) -> [phase_grid_pll]
  FHT-PLL_simulink/2(omega_grid_fht_pll) -> [omega_grid_pll_pu]
  ug_abc_pu/1 -> FHT-PLL performance/1, FHT-PLL_simulink/1(ug_abc_pu)
  Bus Creator2/1 -> FHT-PLL performance/2
  [omega_grid_pll_pu] -> Bus Creator2/2  "omega_grid_fht_pll"
  [phase_grid_pll] -> Bus Creator2/1  "phase_grid_fht_pll"

== system afe_rst_ctrl/afe_abc_inv_psm_mod1/AFE_control/afe_control/grid_voltage_sequences ==
  Abs : Abs  SaturateOnIntegerOverflow=off
  Demux : Demux
  Demux1 : Demux  Outputs=2
  Saturation : Saturate  UpperLimit=2  LowerLimit=0.1
  Terminator : Terminator
  grid_voltage_sequences1 : afe_uvw_ctrl/grid_voltage_sequences  p=param.afe.uvw
  tag scope: ug_alpha_pu=scoped, ug_beta_pu=scoped, v_grid_neg_eta_avg=scoped, v_grid_neg_xi_avg=scoped, v_grid_pos_eta_avg=scoped, v_grid_pos_xi_avg=scoped
  wires:
  [ugd_abc_pu] -> grid_voltage_sequences1/1
  [phase_grid_pll] -> grid_voltage_sequences1/2
  Abs/1 -> Saturation/1
  [omega_grid_pll_pu] -> Abs/1
  Saturation/1 -> grid_voltage_sequences1/3
  grid_voltage_sequences1/1 -> Demux/1
  Demux/4 -> [v_grid_neg_eta_avg]
  Demux/3 -> [v_grid_neg_xi_avg]
  Demux/2 -> [v_grid_pos_eta_avg]
  Demux/1 -> [v_grid_pos_xi_avg]
  grid_voltage_sequences1/3 -> Demux1/1
  Demux1/1 -> [ug_alpha_pu]
  Demux1/2 -> [ug_beta_pu]
  grid_voltage_sequences1/2 -> Terminator/1

== system afe_rst_ctrl/afe_abc_inv_psm_mod1/AFE_control/afe_control/i_xi_ref ==
  Constant1 : Constant  Value=param.afe.ref.ixi_ref_mod1
  Constant2 : Constant  Value=0
  Delay : Delay  DelayLength=floor(0.25/param.glb_time.ts_afe)
  Switch : Switch  Criteria=u2 > Threshold  SaturateOnIntegerOverflow=off  InputSameDT=off
  Switch1 : Switch  Criteria=u2 > Threshold  SaturateOnIntegerOverflow=off  InputSameDT=off
  Variant Source : VariantSource  VariantControls={false, true}
  discrete-time-low-pass-filter : discrete_time_low_pass_filter/discrete-time-low-pass-filter  tau=0.125  ts=param.glb_time.ts_afe
  i_xi_ref : Outport
  wires:
  Constant1/1 -> Switch/3  "i_xi_ref"
  Constant2/1 -> Switch/1
  [pwr_lim_enable] -> Switch/2
  [pwr_lim_enable] -> Delay/1
  Switch/1 -> discrete-time-low-pass-filter/1, Variant Source/2, Switch1/3
  Delay/1 -> Switch1/2
  discrete-time-low-pass-filter/1 -> Switch1/1
  Switch1/1 -> Variant Source/1
  Variant Source/1 -> i_xi_ref/1

== system afe_rst_ctrl/afe_abc_inv_psm_mod1/AFE_control/afe_control/ig afe quantizzation and one step delay ==
  ig_abc_pu : Inport
  Demux1 : Demux  Outputs=3
  Mux1 : Mux  Inputs=3
  ig afe quantizzation and one step delay : Subsystem
  igd_abc_pu : Outport
  wires:
  Demux1/1 -> ig afe quantizzation and one step delay/1(ig_u_pu)
  Demux1/2 -> ig afe quantizzation and one step delay/2(ig_v_pu)
  ig_abc_pu/1 -> Demux1/1
  Mux1/1 -> igd_abc_pu/1
  Demux1/3 -> ig afe quantizzation and one step delay/3(ig_w_pu)
  ig afe quantizzation and one step delay/2(igd_v_pu) -> Mux1/2
  ig afe quantizzation and one step delay/1(igd_u_pu) -> Mux1/1
  ig afe quantizzation and one step delay/3(igd_w_pu) -> Mux1/3
